simulink model "tdsp_model_wrapper"  (R2025a)
settings: Solver=FixedStepDiscrete  StartTime=0.0  StopTime=T_sim  FixedStep=1/48000  RelTol=1e-3
undefined symbols (not defined in the file or in its folder): T_ch
settings Model: FPTShortcutValueString='{{},{''BaselineRun'',1,1,1,''BaselineRun'','''',{'':26''},''M'',''D'','''','''',{},''M'',''D'',''''},{''EmbeddedRun'',1,1,1,''EmbeddedRun'','''',{'':26''},''M'','''','''','''',{},''M'','''',''''},{''EmbeddedRun_2'',1,1,1,''EmbeddedRun_2'','''',{'':26''},''M'','''','''','''',{},''M'','''',''''},{''BaselineRun_2'',1,1,1,''BaselineRun_2'','''',{'':26''},''M'',''D'','''','''',{},''M'',''D'',''''},{''EmbeddedRun_3'',1,1,1,''EmbeddedRun_3'','''',{'':26''},''M'','''','''','''',{},''M'','''',''''}}'  Creator=eoencue1  LastModifiedBy=eoencue1
settings OptimizationCC: DefaultParameterBehavior=Inlined  EnhancedBackFolding=on  PassReuseOutputArgsAs=Individual arguments  OptimizeBlockOrder=speed  DifferentSizesBufferReuse=on  OptimizationCustomize=off  EfficientTunableParamExpr=on
settings DebuggingCC: SignalRangeChecking=warning  ParameterTunabilityLossMsg=error
settings HardwareCC: ProdBitPerPointer=32.0  ProdBitPerSizeT=32.0  ProdBitPerPtrDiffT=32.0  ProdLargestAtomicFloat=None  ProdWordSize=32.0  ProdLongLongMode=on  ProdHWDeviceType=Custom Processor->Custom
settings ModelReferenceCC: ModelReferenceNumInstancesAllowed=Single
settings SFSimCC: MATLABDynamicMemAlloc=off
settings RTWCC: SystemTargetFile=ert.tlc  GenCodeOnly=on  TemplateMakefile=ert_default_tmf  Description=Embedded Coder
settings CodeAppCC: ForceParamTrailComments=on  IgnoreCustomStorageClasses=off  OperatorAnnotations=on  SimulinkDataObjDesc=on  SFDataObjDesc=on  InsertBlockDesc=on
settings ERTTargetCC: ExtModeTransport=0.0  ExtModeStaticAlloc=off  ExtModeMexFile=ext_comm  ExtModeIntrfLevel=Level1  ERTCustomFileTemplate=example_file_process.tlc  TargetLangStandard=C99 (ISO)  SubcomponentCodeInterfacePackaging=Nonreusable function  SupportNonFinite=off

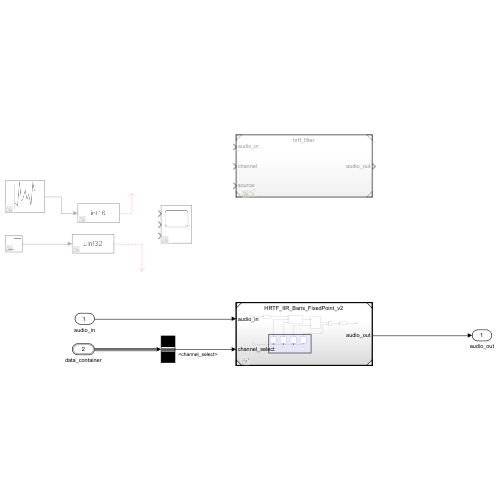
[thumbnail: Simulink's stored preview of the top-level diagram]
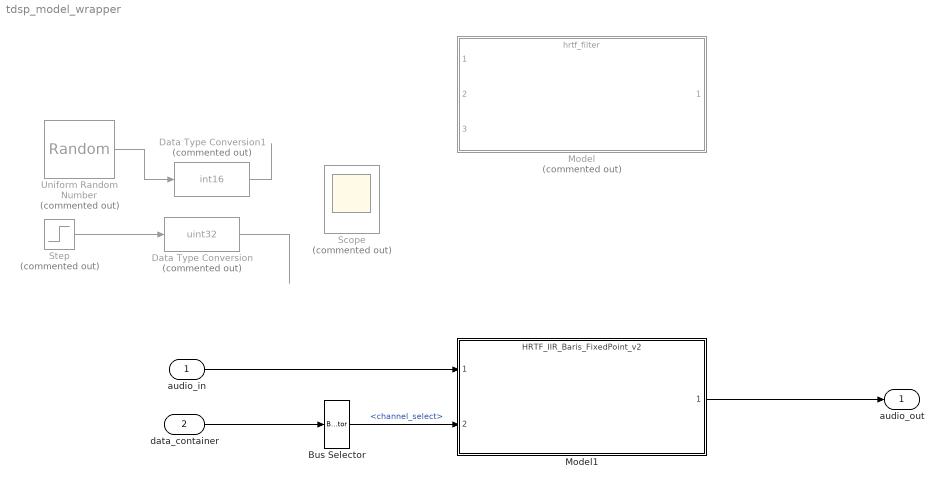
== system tdsp_model_wrapper ==
  audio_in : Inport  OutDataTypeStr=int16  SampleTime=1/48000
  data_container : Inport  Port=2  OutDataTypeStr=Bus: tdsp_data_container  SampleTime=1/48000
  Bus Selector : BusSelector  OutputSignals=channel_select
  Data Type Conversion : DataTypeConversion  Commented=on  OutDataTypeStr=uint32  SaturateOnIntegerOverflow=off  RndMeth=Floor
  Data Type Conversion1 : DataTypeConversion  Commented=on  OutDataTypeStr=int16  RndMeth=Floor
  Model : ModelReference  Commented=on  ModelNameDialog=hrtf_filter.slx  SimulationMode=Normal  ModelReferenceVersion=1.33
  Model1 : ModelReference  ModelNameDialog=HRTF_IIR_Baris_FixedPoint_v2.slx  SimulationMode=Normal  ModelReferenceVersion=1.27
  Scope : Scope  Commented=on  NumInputPorts=3
      settings: ActiveDisplayYMinimum=-34630.2049875089  ActiveDisplayYMaximum=41367.142690723507
  Step : Step  Commented=on  Time=T_ch  SampleTime=1/48000
  Uniform Random Number : UniformRandomNumber  Commented=on  Minimum=-32768  Maximum=32767  SampleTime=1/48000
  audio_out : Outport  OutDataTypeStr=int16  SampleTime=1/48000
  wires:
  audio_in/1 -> Model1/1
  data_container/1 -> Bus Selector/1
  Bus Selector/1 -> Model1/2  "<channel_select>"
  Model1/1 -> audio_out/1
  Uniform Random Number/1 -> Data Type Conversion1/1
  Step/1 -> Data Type Conversion/1
  Data Type Conversion/1 -> ?
  Data Type Conversion1/1 -> ?
